simulink model "MVC27_Sim"  (R2022b)
settings: Solver=FixedStepAuto  StartTime=0.0  StopTime=Sim.Tsim  FixedStep=Sim.Ts  RelTol=1e-3
values from neighbouring files (symbols this model uses):
  g = 9.81    [sim_para.m]
  tdis_FL = 0.3455    [meso_para.m]
  tdis_FR = 0.3455    [meso_para.m]
  tdis_RL = 1 - (tdis_FR + tdis_FL + tdis_RR)    (= 0.1545)    [meso_para.m]
  tdis_RR = 0.1545    [meso_para.m]
undefined symbols (not defined in the file or in its folder): Ctl, DYC, EPS, flag, Motor, Road, Sim, Slip, Steer, Vehicle, Wheel, Wind, WPT
libraries: simulink x3
(part 2 of 2)

== system MVC27_Sim/Energy Management & Motion Control Strategy/Steer angle and yaw moment control/steering angle control ==
  POS_Y : Inport
  Yaw : Inport  Port=2
  Add : Sum  Inputs=+-
  Add1 : Sum  Inputs=+-
  Add2 : Sum
  Constant : Constant  Value=0
  Constant1 : Constant  Value=0
  Position control gain : Gain  Gain=Steer.Kp_pos
  Yaw control gain : Gain  Gain=Steer.Kp_yaw
  delta_f_cmd : Outport
  wires:
  Constant/1 -> Add/1
  POS_Y/1 -> Add/2
  Add/1 -> Position control gain/1
  Constant1/1 -> Add1/1
  Yaw/1 -> Add1/2
  Add1/1 -> Yaw control gain/1
  Position control gain/1 -> Add2/1
  Yaw control gain/1 -> Add2/2
  Add2/1 -> delta_f_cmd/1

== system MVC27_Sim/Energy Management & Motion Control Strategy/Steer angle and yaw moment control/yaw moment control_pos_y ==
  In1 : Inport
  Add : Sum  Inputs=+-
  Add1 : Sum  Inputs=+++
  Constant : Constant  Value=0
  Gain1 : Gain  Gain=DYC.Kd_pos
  Gain2 : Gain  Gain=DYC.Kp_pos
  Gain3 : Gain  Gain=DYC.Ki_pos
  Integrator : Integrator
  Transfer Fcn : TransferFcn  Numerator=[1 0]  Denominator=[DYC.Taud_pos 1]
  Out1 : Outport
  wires:
  Gain2/1 -> Add1/1
  Add1/1 -> Out1/1
  Integrator/1 -> Add1/2
  Transfer Fcn/1 -> Add1/3
  Gain1/1 -> Transfer Fcn/1
  Gain3/1 -> Integrator/1
  Constant/1 -> Add/1
  Add/1 -> Gain1/1, Gain2/1, Gain3/1
  In1/1 -> Add/2

== system MVC27_Sim/Energy Management & Motion Control Strategy/Steer angle and yaw moment control/yaw moment control_yaw ==
  In1 : Inport
  Add : Sum  Inputs=+-
  Constant : Constant  Value=0
  Gain3 : Gain  Gain=DYC.Kp_yaw
  Out1 : Outport
  wires:
  Gain3/1 -> Out1/1
  Constant/1 -> Add/1
  Add/1 -> Gain3/1
  In1/1 -> Add/2

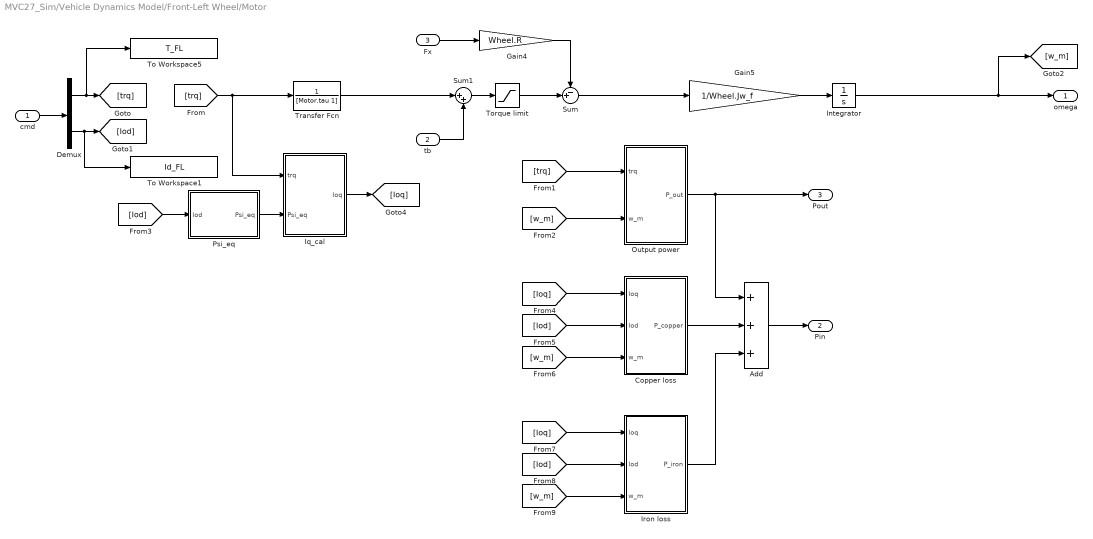
== system MVC27_Sim/Vehicle Dynamics Model/Front-Left Wheel/Motor ==
  cmd : Inport
  tb : Inport  Port=2
  Fx : Inport  Port=3
  Add : Sum  Inputs=+++
  Copper loss : Subsystem
  Demux : Demux  Outputs=2
  Gain4 : Gain  Gain=Wheel.R  SaturateOnIntegerOverflow=on  OutDataTypeStr=Inherit: Same as input  ParamDataTypeStr=Inherit: Same as input
  Gain5 : Gain  Gain=1/Wheel.Jw_f  SaturateOnIntegerOverflow=on  OutDataTypeStr=Inherit: Same as input  ParamDataTypeStr=Inherit: Same as input
  Integrator : Integrator  InitialCondition=Sim.Ini_W  LowerSaturationLimit=0
  Iq_cal : Subsystem
  Iron loss : Subsystem
  Output power : Subsystem
  Psi_eq : Subsystem
  Sum : Sum  Inputs=-+|  SaturateOnIntegerOverflow=on
  Sum1 : Sum  Inputs=|++
  To Workspace1 : ToWorkspace  VariableName=Id_FL  SampleTime=-1
  To Workspace5 : ToWorkspace  VariableName=T_FL  SampleTime=-1
  Torque limit : Saturate  UpperLimit=Motor.Tmax_f  LowerLimit=-Motor.Tmax_f
  Transfer Fcn : TransferFcn  Denominator=[Motor.tau 1]
  omega : Outport
  Pin : Outport  Port=2
  Pout : Outport  Port=3
  wires:
  Gain4/1 -> Sum/1
  Gain5/1 -> Integrator/1
  Sum/1 -> Gain5/1
  Torque limit/1 -> Sum/2
  cmd/1 -> Demux/1
  Demux/1 -> To Workspace5/1, [trq]
  Sum1/1 -> Torque limit/1
  tb/1 -> Sum1/2
  Demux/2 -> To Workspace1/1, [Iod]
  Fx/1 -> Gain4/1
  [trq] -> Output power/1(trq)
  [w_m] -> Output power/2(w_m)
  Iq_cal/1(Ioq) -> [Ioq]
  [Iod] -> Psi_eq/1(Iod)
  Psi_eq/1(Psi_eq) -> Iq_cal/2(Psi_eq)
  [Ioq] -> Copper loss/1(Ioq)
  [Iod] -> Copper loss/2(Iod)
  [w_m] -> Copper loss/3(w_m)
  [Ioq] -> Iron loss/1(Ioq)
  [Iod] -> Iron loss/2(Iod)
  [w_m] -> Iron loss/3(w_m)
  Copper loss/1(P_copper) -> Add/2
  Output power/1(P_out) -> Pout/1, Add/1
  Iron loss/1(P_iron) -> Add/3
  Add/1 -> Pin/1
  Integrator/1 -> omega/1, [w_m]
  [trq] -> Transfer Fcn/1, Iq_cal/1(trq)
  Transfer Fcn/1 -> Sum1/1

== system MVC27_Sim/Vehicle Dynamics Model/Front-Left Wheel/Tire force model ==
  V : Inport
  Vw : Inport  Port=2
  alpha : Inport  Port=3
  mu : Inport  Port=4
  Fz : Inport  Port=5
  Demux : Demux  Outputs=3
      settings: DisplayOption=none
  Level-2 MATLAB S-Function : M-S-Function  FunctionName=LambdaMethod
  Mux : Mux  Inputs=5
  Slip ratio calculation : Subsystem
  Transfer Fcn : TransferFcn  Denominator=[0.01 1]
  Transfer Fcn1 : TransferFcn  Denominator=[0.01 1]
  Transfer Fcn2 : TransferFcn  Denominator=[0.01 1]
  lambda_cal : Scope
  Fx : Outport
  Fy : Outport  Port=2
  lambda : Outport  Port=3
  wires:
  V/1 -> Slip ratio calculation/1(V), Mux/1
  Demux/2 -> Transfer Fcn1/1
  Demux/3 -> Transfer Fcn2/1
  Vw/1 -> Slip ratio calculation/2(Vw), Mux/2
  Mux/1 -> Level-2 MATLAB S-Function/1
  mu/1 -> Mux/4
  Demux/1 -> Transfer Fcn/1
  Fz/1 -> Mux/5
  alpha/1 -> Mux/3
  Slip ratio calculation/1(lambda) -> lambda_cal/1
  Transfer Fcn/1 -> Fx/1
  Transfer Fcn1/1 -> Fy/1
  Transfer Fcn2/1 -> lambda/1
  Level-2 MATLAB S-Function/1 -> Demux/1

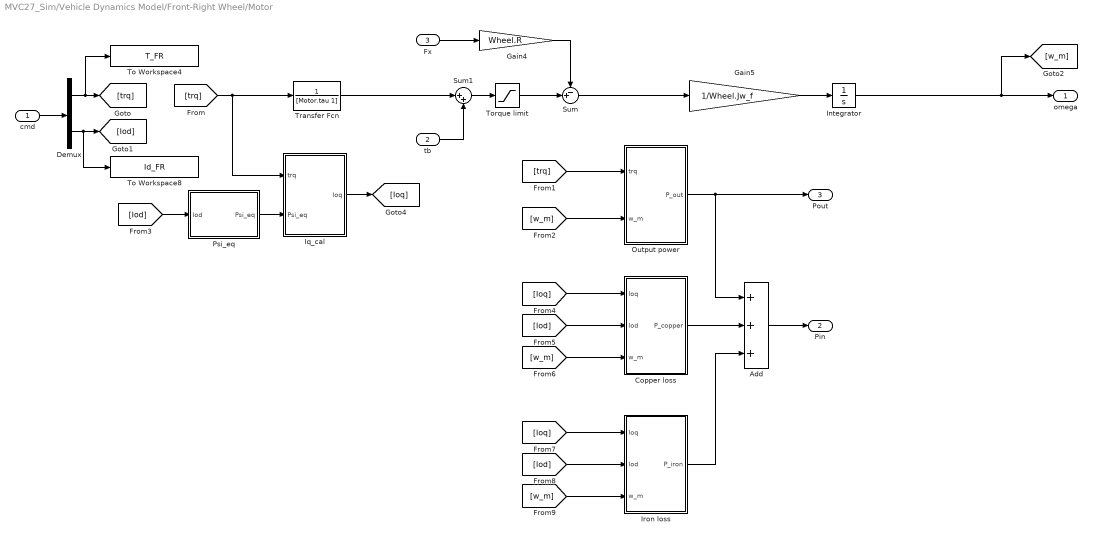
== system MVC27_Sim/Vehicle Dynamics Model/Front-Right Wheel/Motor ==
  cmd : Inport
  tb : Inport  Port=2
  Fx : Inport  Port=3
  Add : Sum  Inputs=+++
  Copper loss : Subsystem
  Demux : Demux  Outputs=2
  Gain4 : Gain  Gain=Wheel.R  SaturateOnIntegerOverflow=on  OutDataTypeStr=Inherit: Same as input  ParamDataTypeStr=Inherit: Same as input
  Gain5 : Gain  Gain=1/Wheel.Jw_f  SaturateOnIntegerOverflow=on  OutDataTypeStr=Inherit: Same as input  ParamDataTypeStr=Inherit: Same as input
  Integrator : Integrator  InitialCondition=Sim.Ini_W  LowerSaturationLimit=0
  Iq_cal : Subsystem
  Iron loss : Subsystem
  Output power : Subsystem
  Psi_eq : Subsystem
  Sum : Sum  Inputs=-+|  SaturateOnIntegerOverflow=on
  Sum1 : Sum  Inputs=|++
  To Workspace4 : ToWorkspace  VariableName=T_FR  SampleTime=-1
  To Workspace8 : ToWorkspace  VariableName=Id_FR  SampleTime=-1
  Torque limit : Saturate  UpperLimit=Motor.Tmax_f  LowerLimit=-Motor.Tmax_f
  Transfer Fcn : TransferFcn  Denominator=[Motor.tau 1]
  omega : Outport
  Pin : Outport  Port=2
  Pout : Outport  Port=3
  wires:
  Gain4/1 -> Sum/1
  Gain5/1 -> Integrator/1
  Sum/1 -> Gain5/1
  Torque limit/1 -> Sum/2
  cmd/1 -> Demux/1
  Demux/1 -> To Workspace4/1, [trq]
  Sum1/1 -> Torque limit/1
  tb/1 -> Sum1/2
  Demux/2 -> To Workspace8/1, [Iod]
  Fx/1 -> Gain4/1
  [trq] -> Output power/1(trq)
  [w_m] -> Output power/2(w_m)
  Iq_cal/1(Ioq) -> [Ioq]
  [Iod] -> Psi_eq/1(Iod)
  Psi_eq/1(Psi_eq) -> Iq_cal/2(Psi_eq)
  [Ioq] -> Copper loss/1(Ioq)
  [Iod] -> Copper loss/2(Iod)
  [w_m] -> Copper loss/3(w_m)
  [Ioq] -> Iron loss/1(Ioq)
  [Iod] -> Iron loss/2(Iod)
  [w_m] -> Iron loss/3(w_m)
  Copper loss/1(P_copper) -> Add/2
  Output power/1(P_out) -> Pout/1, Add/1
  Iron loss/1(P_iron) -> Add/3
  Add/1 -> Pin/1
  Integrator/1 -> omega/1, [w_m]
  [trq] -> Transfer Fcn/1, Iq_cal/1(trq)
  Transfer Fcn/1 -> Sum1/1

== system MVC27_Sim/Vehicle Dynamics Model/Front-Right Wheel/Tire force model ==
  V : Inport
  Vw : Inport  Port=2
  alpha : Inport  Port=3
  mu : Inport  Port=4
  Fz : Inport  Port=5
  Demux : Demux  Outputs=3
      settings: DisplayOption=none
  Level-2 MATLAB S-Function : M-S-Function  FunctionName=LambdaMethod
  Mux : Mux  Inputs=5
  Slip ratio calculation : Subsystem
  Transfer Fcn : TransferFcn  Denominator=[0.01 1]
  Transfer Fcn1 : TransferFcn  Denominator=[0.01 1]
  Transfer Fcn2 : TransferFcn  Denominator=[0.01 1]
  lambda_cal : Scope
  Fx : Outport
  Fy : Outport  Port=2
  lambda : Outport  Port=3
  wires:
  V/1 -> Slip ratio calculation/1(V), Mux/1
  Demux/2 -> Transfer Fcn1/1
  Demux/3 -> Transfer Fcn2/1
  Vw/1 -> Slip ratio calculation/2(Vw), Mux/2
  Mux/1 -> Level-2 MATLAB S-Function/1
  mu/1 -> Mux/4
  Demux/1 -> Transfer Fcn/1
  Fz/1 -> Mux/5
  alpha/1 -> Mux/3
  Slip ratio calculation/1(lambda) -> lambda_cal/1
  Transfer Fcn/1 -> Fx/1
  Transfer Fcn1/1 -> Fy/1
  Transfer Fcn2/1 -> lambda/1
  Level-2 MATLAB S-Function/1 -> Demux/1

== system MVC27_Sim/Vehicle Dynamics Model/Rear-Left Wheel/Motor ==
  cmd : Inport
  tb : Inport  Port=2
  Fx : Inport  Port=3
  Add : Sum  Inputs=+++
  Copper loss : Subsystem
  Demux : Demux  Outputs=2
  Gain4 : Gain  Gain=Wheel.R  SaturateOnIntegerOverflow=on  OutDataTypeStr=Inherit: Same as input  ParamDataTypeStr=Inherit: Same as input
  Gain5 : Gain  Gain=1/Wheel.Jw_r  SaturateOnIntegerOverflow=on  OutDataTypeStr=Inherit: Same as input  ParamDataTypeStr=Inherit: Same as input
  Integrator : Integrator  InitialCondition=Sim.Ini_W  LowerSaturationLimit=0
  Iq_cal : Subsystem
  Iron loss : Subsystem
  Output power : Subsystem
  Psi_eq : Subsystem
  Sum : Sum  Inputs=-+|  SaturateOnIntegerOverflow=on
  Sum1 : Sum  Inputs=|++
  To Workspace3 : ToWorkspace  VariableName=Id_RL  SampleTime=-1
  To Workspace7 : ToWorkspace  VariableName=T_RL  SampleTime=-1
  Torque limit : Saturate  UpperLimit=Motor.Tmax_r  LowerLimit=-Motor.Tmax_r
  Transfer Fcn : TransferFcn  Denominator=[Motor.tau 1]
  omega : Outport
  Pin : Outport  Port=2
  Pout : Outport  Port=3
  wires:
  Gain4/1 -> Sum/1
  Gain5/1 -> Integrator/1
  Sum/1 -> Gain5/1
  Torque limit/1 -> Sum/2
  cmd/1 -> Demux/1
  Demux/1 -> To Workspace7/1, [trq]
  [trq] -> Transfer Fcn/1, Iq_cal/1(trq)
  Sum1/1 -> Torque limit/1
  tb/1 -> Sum1/2
  Demux/2 -> To Workspace3/1, [Iod]
  Fx/1 -> Gain4/1
  [trq] -> Output power/1(trq)
  [w_m] -> Output power/2(w_m)
  Iq_cal/1(Ioq) -> [Ioq]
  [Iod] -> Psi_eq/1(Iod)
  Psi_eq/1(Psi_eq) -> Iq_cal/2(Psi_eq)
  [Ioq] -> Copper loss/1(Ioq)
  [Iod] -> Copper loss/2(Iod)
  [w_m] -> Copper loss/3(w_m)
  [Ioq] -> Iron loss/1(Ioq)
  [Iod] -> Iron loss/2(Iod)
  [w_m] -> Iron loss/3(w_m)
  Copper loss/1(P_copper) -> Add/2
  Output power/1(P_out) -> Pout/1, Add/1
  Iron loss/1(P_iron) -> Add/3
  Add/1 -> Pin/1
  Integrator/1 -> omega/1, [w_m]
  Transfer Fcn/1 -> Sum1/1

== system MVC27_Sim/Vehicle Dynamics Model/Rear-Left Wheel/Tire force model ==
  V : Inport
  Vw : Inport  Port=2
  alpha : Inport  Port=3
  mu : Inport  Port=4
  Fz : Inport  Port=5
  Demux : Demux  Outputs=3
      settings: DisplayOption=none
  Level-2 MATLAB S-Function : M-S-Function  FunctionName=LambdaMethod
  Mux : Mux  Inputs=5
  Slip ratio calculation : Subsystem
  Transfer Fcn : TransferFcn  Denominator=[0.01 1]
  Transfer Fcn1 : TransferFcn  Denominator=[0.01 1]
  Transfer Fcn2 : TransferFcn  Denominator=[0.01 1]
  lambda_cal : Scope
  Fx : Outport
  Fy : Outport  Port=2
  lambda : Outport  Port=3
  wires:
  V/1 -> Slip ratio calculation/1(V), Mux/1
  Demux/3 -> Transfer Fcn2/1
  Vw/1 -> Slip ratio calculation/2(Vw), Mux/2
  mu/1 -> Mux/4
  Demux/1 -> Transfer Fcn/1
  Fz/1 -> Mux/5
  alpha/1 -> Mux/3
  Slip ratio calculation/1(lambda) -> lambda_cal/1
  Demux/2 -> Transfer Fcn1/1
  Transfer Fcn/1 -> Fx/1
  Transfer Fcn1/1 -> Fy/1
  Transfer Fcn2/1 -> lambda/1
  Mux/1 -> Level-2 MATLAB S-Function/1
  Level-2 MATLAB S-Function/1 -> Demux/1

== system MVC27_Sim/Vehicle Dynamics Model/Rear-Right Wheel/Motor ==
  cmd : Inport
  tb : Inport  Port=2
  Fx : Inport  Port=3
  Add : Sum  Inputs=+++
  Copper loss : Subsystem
  Demux : Demux  Outputs=2
  Gain4 : Gain  Gain=Wheel.R  SaturateOnIntegerOverflow=on  OutDataTypeStr=Inherit: Same as input  ParamDataTypeStr=Inherit: Same as input
  Gain5 : Gain  Gain=1/Wheel.Jw_r  SaturateOnIntegerOverflow=on  OutDataTypeStr=Inherit: Same as input  ParamDataTypeStr=Inherit: Same as input
  Integrator : Integrator  InitialCondition=Sim.Ini_W  LowerSaturationLimit=0
  Iq_cal : Subsystem
  Iron loss : Subsystem
  Output power : Subsystem
  Psi_eq : Subsystem
  Sum : Sum  Inputs=-+|  SaturateOnIntegerOverflow=on
  Sum1 : Sum  Inputs=|++
  To Workspace2 : ToWorkspace  VariableName=Id_RR  SampleTime=-1
  To Workspace6 : ToWorkspace  VariableName=T_RR  SampleTime=-1
  Torque limit : Saturate  UpperLimit=Motor.Tmax_r  LowerLimit=-Motor.Tmax_r
  Transfer Fcn : TransferFcn  Denominator=[Motor.tau 1]
  omega : Outport
  Pin : Outport  Port=2
  Pout : Outport  Port=3
  wires:
  Gain4/1 -> Sum/1
  Gain5/1 -> Integrator/1
  Sum/1 -> Gain5/1
  Torque limit/1 -> Sum/2
  cmd/1 -> Demux/1
  Demux/1 -> To Workspace6/1, [trq]
  Sum1/1 -> Torque limit/1
  tb/1 -> Sum1/2
  Demux/2 -> To Workspace2/1, [Iod]
  Fx/1 -> Gain4/1
  [trq] -> Output power/1(trq)
  [w_m] -> Output power/2(w_m)
  Iq_cal/1(Ioq) -> [Ioq]
  [Iod] -> Psi_eq/1(Iod)
  Psi_eq/1(Psi_eq) -> Iq_cal/2(Psi_eq)
  [Ioq] -> Copper loss/1(Ioq)
  [Iod] -> Copper loss/2(Iod)
  [w_m] -> Copper loss/3(w_m)
  [Ioq] -> Iron loss/1(Ioq)
  [Iod] -> Iron loss/2(Iod)
  [w_m] -> Iron loss/3(w_m)
  Copper loss/1(P_copper) -> Add/2
  Output power/1(P_out) -> Pout/1, Add/1
  Iron loss/1(P_iron) -> Add/3
  Add/1 -> Pin/1
  Integrator/1 -> omega/1, [w_m]
  [trq] -> Transfer Fcn/1, Iq_cal/1(trq)
  Transfer Fcn/1 -> Sum1/1

== system MVC27_Sim/Vehicle Dynamics Model/Rear-Right Wheel/Tire force model ==
  V : Inport
  Vw : Inport  Port=2
  alpha : Inport  Port=3
  mu : Inport  Port=4
  Fz : Inport  Port=5
  Demux : Demux  Outputs=3
      settings: DisplayOption=none
  Level-2 MATLAB S-Function : M-S-Function  FunctionName=LambdaMethod
  Mux : Mux  Inputs=5
  Slip ratio calculation : Subsystem
  Transfer Fcn : TransferFcn  Denominator=[0.01 1]
  Transfer Fcn1 : TransferFcn  Denominator=[0.01 1]
  Transfer Fcn2 : TransferFcn  Denominator=[0.01 1]
  lambda_cal : Scope
  Fx : Outport
  Fy : Outport  Port=2
  lambda : Outport  Port=3
  wires:
  V/1 -> Slip ratio calculation/1(V), Mux/1
  Demux/2 -> Transfer Fcn1/1
  Demux/3 -> Transfer Fcn2/1
  Vw/1 -> Slip ratio calculation/2(Vw), Mux/2
  Mux/1 -> Level-2 MATLAB S-Function/1
  mu/1 -> Mux/4
  Demux/1 -> Transfer Fcn/1
  Fz/1 -> Mux/5
  alpha/1 -> Mux/3
  Slip ratio calculation/1(lambda) -> lambda_cal/1
  Transfer Fcn/1 -> Fx/1
  Transfer Fcn1/1 -> Fy/1
  Transfer Fcn2/1 -> lambda/1
  Level-2 MATLAB S-Function/1 -> Demux/1

== system MVC27_Sim/Vehicle Dynamics Model/Vehicle Body/Condition to prevent division by zero ==
  In : Inport
  Constant : Constant  Value=0.1
  Scope : Scope
  Switch : Switch  Criteria=u2 > Threshold  Threshold=0.1  SaturateOnIntegerOverflow=off  InputSameDT=off
  Out : Outport
  wires:
  In/1 -> Switch/1, Switch/2
  Constant/1 -> Switch/3
  Switch/1 -> Scope/1, Out/1

== system MVC27_Sim/Vehicle Dynamics Model/Vehicle Body/Driving resistance ==
  Vx : Inport
  Abs : Abs  SaturateOnIntegerOverflow=off
  Air resistance : Constant  Value=1/2*Vehicle.rho*Vehicle.Cd*Vehicle.Afpa
  Memory1 : Memory  InheritSampleTime=on  LinearizeMemory=on
  Plus1 : Sum
  Product : Product  Inputs=3
  Rolling resistance : Constant  Value=Vehicle.mu0*Vehicle.M*g
  DR : Outport
  wires:
  Product/1 -> Plus1/2
  Air resistance/1 -> Product/1
  Plus1/1 -> DR/1
  Vx/1 -> Memory1/1
  Memory1/1 -> Product/2, Abs/1
  Abs/1 -> Product/3
  Rolling resistance/1 -> Plus1/1

== system MVC27_Sim/Vehicle Dynamics Model/Vehicle Body/Lateral disturbance ==
  Wind_flag : Inport
  Clock{,1..3} (4 alike) : Clock
  Product : Product
  Product1 : Product
  Switch : Switch  Criteria=u2 > Threshold  Threshold=Wind.time_start  SaturateOnIntegerOverflow=off  InputSameDT=off
  Switch1 : Switch  Criteria=u2 > Threshold  Threshold=Wind.time_stop  SaturateOnIntegerOverflow=off  InputSameDT=off
  Switch2 : Switch  Criteria=u2 > Threshold  Threshold=Wind.time_start  SaturateOnIntegerOverflow=off  InputSameDT=off
  Switch3 : Switch  Criteria=u2 > Threshold  Threshold=Wind.time_stop  SaturateOnIntegerOverflow=off  InputSameDT=off
  Wind force : Scope
  Wind force.No : Constant  Value=0
  Wind force.Yes : Constant  Value=Wind.force
  Wind moment : Scope
  Wind moment.No : Constant  Value=0
  Wind moment.Yes : Constant  Value=Wind.moment
  Nzd : Outport
  Fyd : Outport  Port=2
  wires:
  Clock/1 -> Switch/2
  Clock1/1 -> Switch1/2
  Wind force.Yes/1 -> Switch/1
  Wind force.No/1 -> Switch1/1, Switch/3
  Switch/1 -> Switch1/3
  Switch2/1 -> Switch3/3
  Clock2/1 -> Switch2/2
  Wind moment.Yes/1 -> Switch2/1
  Clock3/1 -> Switch3/2
  Wind moment.No/1 -> Switch3/1, Switch2/3
  Switch3/1 -> Product/1
  Switch1/1 -> Product1/2
  Product1/1 -> Wind force/1, Fyd/1
  Product/1 -> Wind moment/1, Nzd/1
  Wind_flag/1 -> Product1/1, Product/2

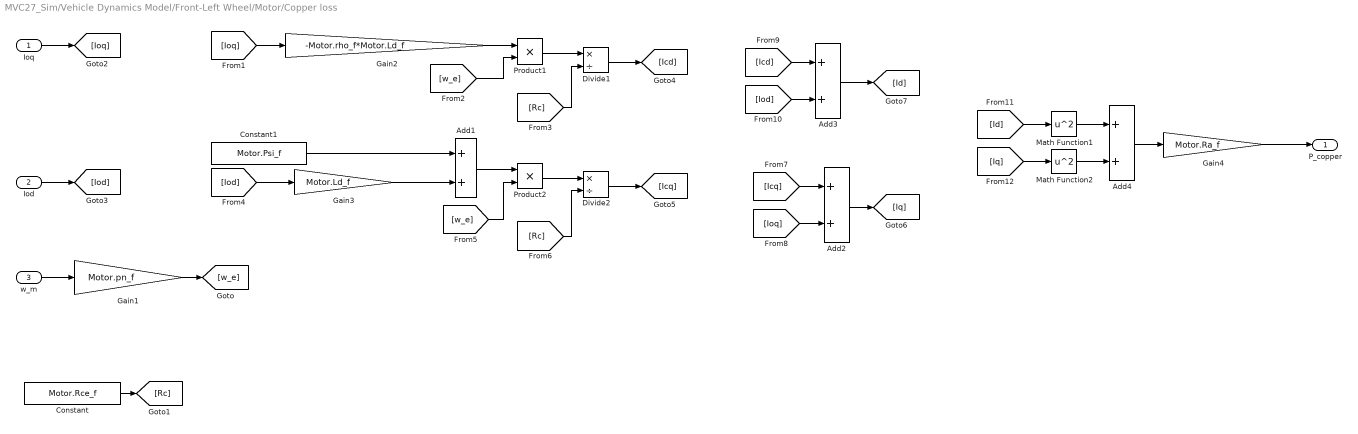
== system MVC27_Sim/Vehicle Dynamics Model/Front-Left Wheel/Motor/Copper loss ==
  Ioq : Inport
  Iod : Inport  Port=2
  w_m : Inport  Port=3
  Add{1..4} (4 alike) : Sum
  Constant : Constant  Value=Motor.Rce_f
  Constant1 : Constant  Value=Motor.Psi_f
  Divide1 : Product  Inputs=*/
  Divide2 : Product  Inputs=*/
  Gain1 : Gain  Gain=Motor.pn_f
  Gain2 : Gain  Gain=-Motor.rho_f*Motor.Ld_f
  Gain3 : Gain  Gain=Motor.Ld_f
  Gain4 : Gain  Gain=Motor.Ra_f
  Math Function1 : Math  Operator=square  SignedPower=on
  Math Function2 : Math  Operator=square  SignedPower=on
  Product1 : Product
  Product2 : Product
  P_copper : Outport
  wires:
  w_m/1 -> Gain1/1
  Gain1/1 -> [w_e]
  Ioq/1 -> [Ioq]
  Iod/1 -> [Iod]
  [Ioq] -> Gain2/1
  Gain2/1 -> Product1/1
  [w_e] -> Product1/2
  Product1/1 -> Divide1/1
  [Rc] -> Divide1/2
  Divide1/1 -> [Icd]
  Constant1/1 -> Add1/1
  [Iod] -> Gain3/1
  Gain3/1 -> Add1/2
  Add1/1 -> Product2/1
  [w_e] -> Product2/2
  Product2/1 -> Divide2/1
  [Rc] -> Divide2/2
  Divide2/1 -> [Icq]
  [Icq] -> Add2/1
  [Ioq] -> Add2/2
  Add2/1 -> [Iq]
  [Icd] -> Add3/1
  Add3/1 -> [Id]
  [Iod] -> Add3/2
  [Id] -> Math Function1/1
  [Iq] -> Math Function2/1
  Math Function1/1 -> Add4/1
  Math Function2/1 -> Add4/2
  Add4/1 -> Gain4/1
  Gain4/1 -> P_copper/1
  Constant/1 -> [Rc]

== system MVC27_Sim/Vehicle Dynamics Model/Front-Left Wheel/Motor/Iq_cal ==
  trq : Inport
  Psi_eq : Inport  Port=2
  Divide : Product  Inputs=*/
  Gain : Gain  Gain=Motor.pn_f
  Ioq : Outport
  wires:
  Gain/1 -> Divide/2
  Divide/1 -> Ioq/1
  Psi_eq/1 -> Gain/1
  trq/1 -> Divide/1

== system MVC27_Sim/Vehicle Dynamics Model/Front-Left Wheel/Motor/Iron loss ==
  Ioq : Inport
  Iod : Inport  Port=2
  w_m : Inport  Port=3
  Add1 : Sum
  Add4 : Sum
  Constant : Constant  Value=Motor.Rce_f
  Constant1 : Constant  Value=Motor.Psi_f
  Divide1 : Product  Inputs=*/
  Divide2 : Product  Inputs=*/
  Gain1 : Gain  Gain=Motor.pn_f
  Gain2 : Gain  Gain=-Motor.rho_f*Motor.Ld_f
  Gain3 : Gain  Gain=Motor.Ld_f
  Math Function1 : Math  Operator=square  SignedPower=on
  Math Function2 : Math  Operator=square  SignedPower=on
  Product1 : Product
  Product2 : Product
  Product3 : Product
  P_iron : Outport
  wires:
  Gain1/1 -> [w_e]
  w_m/1 -> Gain1/1
  [Rc] -> Divide2/2
  Constant1/1 -> Add1/1
  Gain3/1 -> Add1/2
  Add1/1 -> Product2/1
  Divide1/1 -> [Icd]
  Product1/1 -> Divide1/1
  [Iod] -> Gain3/1
  Gain2/1 -> Product1/1
  Divide2/1 -> [Icq]
  [Rc] -> Divide1/2
  [Ioq] -> Gain2/1
  [w_e] -> Product2/2
  [w_e] -> Product1/2
  Product2/1 -> Divide2/1
  Ioq/1 -> [Ioq]
  Iod/1 -> [Iod]
  [Icd] -> Math Function1/1
  Math Function1/1 -> Add4/1
  [Icq] -> Math Function2/1
  Math Function2/1 -> Add4/2
  Add4/1 -> Product3/1
  [Rc] -> Product3/2
  Product3/1 -> P_iron/1
  Constant/1 -> [Rc]

== system MVC27_Sim/Vehicle Dynamics Model/Front-Left Wheel/Motor/Output power ==
  trq : Inport
  w_m : Inport  Port=2
  Product : Product
  P_out : Outport
  wires:
  trq/1 -> Product/1
  w_m/1 -> Product/2
  Product/1 -> P_out/1

== system MVC27_Sim/Vehicle Dynamics Model/Front-Left Wheel/Motor/Psi_eq ==
  Iod : Inport
  Add : Sum
  Constant : Constant  Value=Motor.Psi_f
  Gain4 : Gain  Gain=(1-Motor.rho_f)*Motor.Ld_f  SaturateOnIntegerOverflow=on  OutDataTypeStr=Inherit: Same as input  ParamDataTypeStr=Inherit: Same as input
  Psi_eq : Outport
  wires:
  Iod/1 -> Gain4/1
  Gain4/1 -> Add/2
  Constant/1 -> Add/1
  Add/1 -> Psi_eq/1

== system MVC27_Sim/Vehicle Dynamics Model/Front-Left Wheel/Tire force model/Slip ratio calculation ==
  V : Inport
  Vw : Inport  Port=2
  Divide : Product  Inputs=*/
  Sum : Sum  Inputs=-+
  max calculation : MinMax  Function=max  Inputs=2
  max calculation1 : MinMax  Function=max  Inputs=2
  small number for anti division by zero : Constant  Value=eps
  lambda : Outport
  wires:
  small number for anti division by zero/1 -> max calculation1/2
  Vw/1 -> max calculation/2, Sum/2
  V/1 -> max calculation/1, Sum/1
  Divide/1 -> lambda/1
  max calculation/1 -> max calculation1/1
  max calculation1/1 -> Divide/2
  Sum/1 -> Divide/1

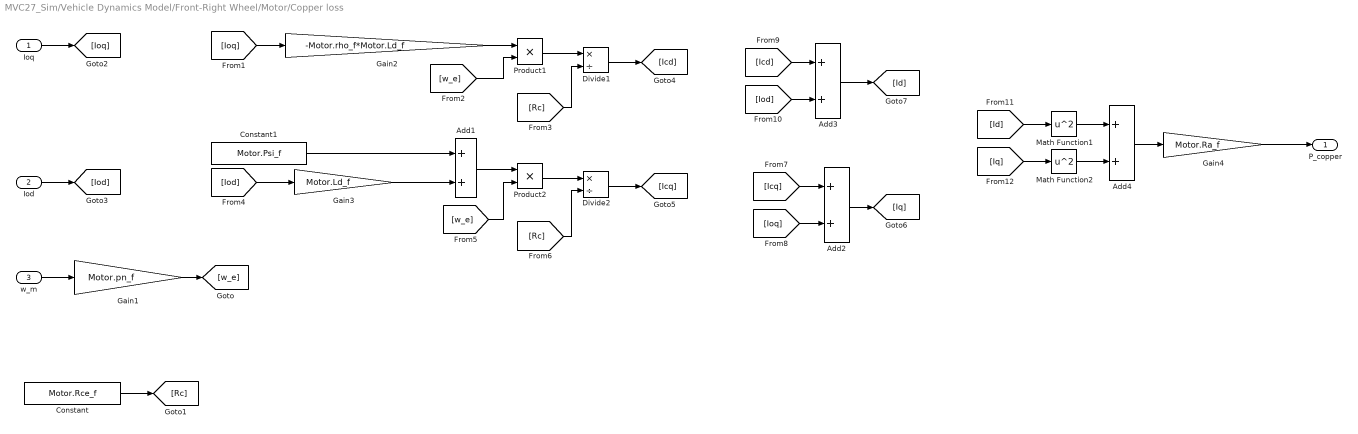
== system MVC27_Sim/Vehicle Dynamics Model/Front-Right Wheel/Motor/Copper loss ==
  Ioq : Inport
  Iod : Inport  Port=2
  w_m : Inport  Port=3
  Add{1..4} (4 alike) : Sum
  Constant : Constant  Value=Motor.Rce_f
  Constant1 : Constant  Value=Motor.Psi_f
  Divide1 : Product  Inputs=*/
  Divide2 : Product  Inputs=*/
  Gain1 : Gain  Gain=Motor.pn_f
  Gain2 : Gain  Gain=-Motor.rho_f*Motor.Ld_f
  Gain3 : Gain  Gain=Motor.Ld_f
  Gain4 : Gain  Gain=Motor.Ra_f
  Math Function1 : Math  Operator=square  SignedPower=on
  Math Function2 : Math  Operator=square  SignedPower=on
  Product1 : Product
  Product2 : Product
  P_copper : Outport
  wires:
  w_m/1 -> Gain1/1
  Gain1/1 -> [w_e]
  Ioq/1 -> [Ioq]
  Iod/1 -> [Iod]
  [Ioq] -> Gain2/1
  Gain2/1 -> Product1/1
  [w_e] -> Product1/2
  Product1/1 -> Divide1/1
  [Rc] -> Divide1/2
  Divide1/1 -> [Icd]
  Constant1/1 -> Add1/1
  [Iod] -> Gain3/1
  Gain3/1 -> Add1/2
  Add1/1 -> Product2/1
  [w_e] -> Product2/2
  Product2/1 -> Divide2/1
  [Rc] -> Divide2/2
  Divide2/1 -> [Icq]
  [Icq] -> Add2/1
  [Ioq] -> Add2/2
  Add2/1 -> [Iq]
  [Icd] -> Add3/1
  Add3/1 -> [Id]
  [Iod] -> Add3/2
  [Id] -> Math Function1/1
  [Iq] -> Math Function2/1
  Math Function1/1 -> Add4/1
  Math Function2/1 -> Add4/2
  Add4/1 -> Gain4/1
  Gain4/1 -> P_copper/1
  Constant/1 -> [Rc]

== system MVC27_Sim/Vehicle Dynamics Model/Front-Right Wheel/Motor/Iq_cal ==
  trq : Inport
  Psi_eq : Inport  Port=2
  Divide : Product  Inputs=*/
  Gain : Gain  Gain=Motor.pn_f
  Ioq : Outport
  wires:
  Psi_eq/1 -> Gain/1
  Gain/1 -> Divide/2
  trq/1 -> Divide/1
  Divide/1 -> Ioq/1

== system MVC27_Sim/Vehicle Dynamics Model/Front-Right Wheel/Motor/Iron loss ==
  Ioq : Inport
  Iod : Inport  Port=2
  w_m : Inport  Port=3
  Add1 : Sum
  Add4 : Sum
  Constant : Constant  Value=Motor.Rce_f
  Constant1 : Constant  Value=Motor.Psi_f
  Divide1 : Product  Inputs=*/
  Divide2 : Product  Inputs=*/
  Gain1 : Gain  Gain=Motor.pn_f
  Gain2 : Gain  Gain=-Motor.rho_f*Motor.Ld_f
  Gain3 : Gain  Gain=Motor.Ld_f
  Math Function1 : Math  Operator=square  SignedPower=on
  Math Function2 : Math  Operator=square  SignedPower=on
  Product1 : Product
  Product2 : Product
  Product3 : Product
  P_iron : Outport
  wires:
  Gain1/1 -> [w_e]
  w_m/1 -> Gain1/1
  [Rc] -> Divide2/2
  Constant1/1 -> Add1/1
  Gain3/1 -> Add1/2
  Add1/1 -> Product2/1
  Divide1/1 -> [Icd]
  Product1/1 -> Divide1/1
  [Iod] -> Gain3/1
  Gain2/1 -> Product1/1
  Divide2/1 -> [Icq]
  [Rc] -> Divide1/2
  [Ioq] -> Gain2/1
  [w_e] -> Product2/2
  [w_e] -> Product1/2
  Product2/1 -> Divide2/1
  Ioq/1 -> [Ioq]
  Iod/1 -> [Iod]
  [Icd] -> Math Function1/1
  Math Function1/1 -> Add4/1
  [Icq] -> Math Function2/1
  Math Function2/1 -> Add4/2
  Add4/1 -> Product3/1
  [Rc] -> Product3/2
  Product3/1 -> P_iron/1
  Constant/1 -> [Rc]

== system MVC27_Sim/Vehicle Dynamics Model/Front-Right Wheel/Motor/Output power ==
  trq : Inport
  w_m : Inport  Port=2
  Product : Product
  P_out : Outport
  wires:
  trq/1 -> Product/1
  w_m/1 -> Product/2
  Product/1 -> P_out/1

== system MVC27_Sim/Vehicle Dynamics Model/Front-Right Wheel/Motor/Psi_eq ==
  Iod : Inport
  Add : Sum
  Constant : Constant  Value=Motor.Psi_f
  Gain4 : Gain  Gain=(1-Motor.rho_f)*Motor.Ld_f  SaturateOnIntegerOverflow=on  OutDataTypeStr=Inherit: Same as input  ParamDataTypeStr=Inherit: Same as input
  Psi_eq : Outport
  wires:
  Iod/1 -> Gain4/1
  Gain4/1 -> Add/2
  Constant/1 -> Add/1
  Add/1 -> Psi_eq/1

== system MVC27_Sim/Vehicle Dynamics Model/Front-Right Wheel/Tire force model/Slip ratio calculation ==
  V : Inport
  Vw : Inport  Port=2
  Divide : Product  Inputs=*/
  Sum : Sum  Inputs=-+
  max calculation : MinMax  Function=max  Inputs=2
  max calculation1 : MinMax  Function=max  Inputs=2
  small number for anti division by zero : Constant  Value=eps
  lambda : Outport
  wires:
  small number for anti division by zero/1 -> max calculation1/2
  Vw/1 -> max calculation/2, Sum/2
  V/1 -> max calculation/1, Sum/1
  Divide/1 -> lambda/1
  max calculation/1 -> max calculation1/1
  max calculation1/1 -> Divide/2
  Sum/1 -> Divide/1

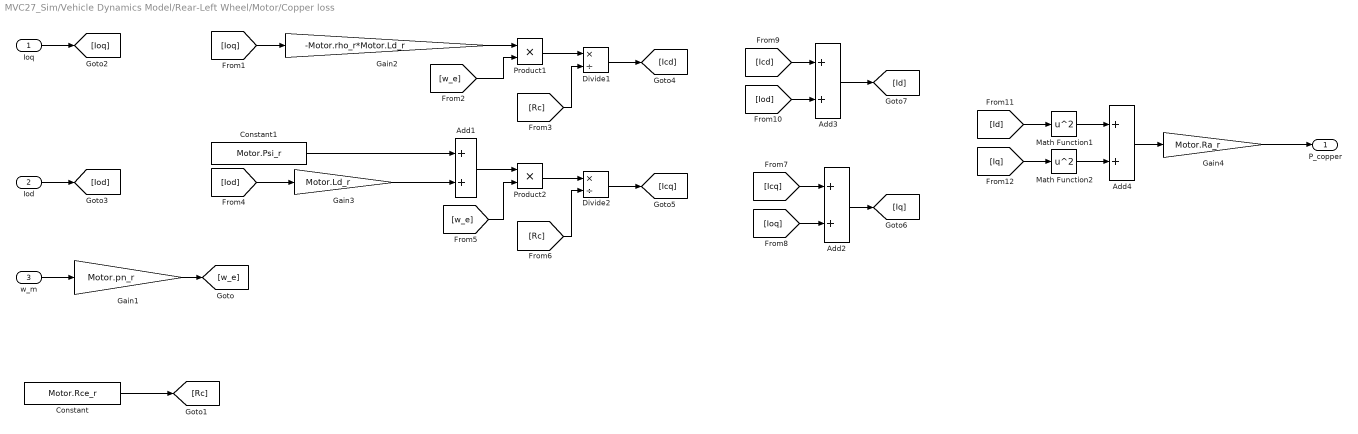
== system MVC27_Sim/Vehicle Dynamics Model/Rear-Left Wheel/Motor/Copper loss ==
  Ioq : Inport
  Iod : Inport  Port=2
  w_m : Inport  Port=3
  Add{1..4} (4 alike) : Sum
  Constant : Constant  Value=Motor.Rce_r
  Constant1 : Constant  Value=Motor.Psi_r
  Divide1 : Product  Inputs=*/
  Divide2 : Product  Inputs=*/
  Gain1 : Gain  Gain=Motor.pn_r
  Gain2 : Gain  Gain=-Motor.rho_r*Motor.Ld_r
  Gain3 : Gain  Gain=Motor.Ld_r
  Gain4 : Gain  Gain=Motor.Ra_r
  Math Function1 : Math  Operator=square  SignedPower=on
  Math Function2 : Math  Operator=square  SignedPower=on
  Product1 : Product
  Product2 : Product
  P_copper : Outport
  wires:
  w_m/1 -> Gain1/1
  Gain1/1 -> [w_e]
  Ioq/1 -> [Ioq]
  Iod/1 -> [Iod]
  [Ioq] -> Gain2/1
  Gain2/1 -> Product1/1
  [w_e] -> Product1/2
  Product1/1 -> Divide1/1
  [Rc] -> Divide1/2
  Divide1/1 -> [Icd]
  Constant1/1 -> Add1/1
  [Iod] -> Gain3/1
  Gain3/1 -> Add1/2
  Add1/1 -> Product2/1
  [w_e] -> Product2/2
  Product2/1 -> Divide2/1
  [Rc] -> Divide2/2
  Divide2/1 -> [Icq]
  [Icq] -> Add2/1
  [Ioq] -> Add2/2
  Add2/1 -> [Iq]
  [Icd] -> Add3/1
  Add3/1 -> [Id]
  [Iod] -> Add3/2
  [Id] -> Math Function1/1
  [Iq] -> Math Function2/1
  Math Function1/1 -> Add4/1
  Math Function2/1 -> Add4/2
  Add4/1 -> Gain4/1
  Gain4/1 -> P_copper/1
  Constant/1 -> [Rc]

== system MVC27_Sim/Vehicle Dynamics Model/Rear-Left Wheel/Motor/Iq_cal ==
  trq : Inport
  Psi_eq : Inport  Port=2
  Divide : Product  Inputs=*/
  Gain : Gain  Gain=Motor.pn_r
  Ioq : Outport
  wires:
  Psi_eq/1 -> Gain/1
  Divide/1 -> Ioq/1
  Gain/1 -> Divide/2
  trq/1 -> Divide/1

== system MVC27_Sim/Vehicle Dynamics Model/Rear-Left Wheel/Motor/Iron loss ==
  Ioq : Inport
  Iod : Inport  Port=2
  w_m : Inport  Port=3
  Add1 : Sum
  Add4 : Sum
  Constant : Constant  Value=Motor.Rce_r
  Constant1 : Constant  Value=Motor.Psi_r
  Divide1 : Product  Inputs=*/
  Divide2 : Product  Inputs=*/
  Gain1 : Gain  Gain=Motor.pn_r
  Gain2 : Gain  Gain=-Motor.rho_r*Motor.Ld_r
  Gain3 : Gain  Gain=Motor.Ld_r
  Math Function1 : Math  Operator=square  SignedPower=on
  Math Function2 : Math  Operator=square  SignedPower=on
  Product1 : Product
  Product2 : Product
  Product3 : Product
  P_iron : Outport
  wires:
  Gain1/1 -> [w_e]
  w_m/1 -> Gain1/1
  [Rc] -> Divide2/2
  Constant1/1 -> Add1/1
  Gain3/1 -> Add1/2
  Add1/1 -> Product2/1
  Divide1/1 -> [Icd]
  Product1/1 -> Divide1/1
  [Iod] -> Gain3/1
  Gain2/1 -> Product1/1
  Divide2/1 -> [Icq]
  [Rc] -> Divide1/2
  [Ioq] -> Gain2/1
  [w_e] -> Product2/2
  [w_e] -> Product1/2
  Product2/1 -> Divide2/1
  Ioq/1 -> [Ioq]
  Iod/1 -> [Iod]
  [Icd] -> Math Function1/1
  Math Function1/1 -> Add4/1
  [Icq] -> Math Function2/1
  Math Function2/1 -> Add4/2
  Add4/1 -> Product3/1
  [Rc] -> Product3/2
  Product3/1 -> P_iron/1
  Constant/1 -> [Rc]

== system MVC27_Sim/Vehicle Dynamics Model/Rear-Left Wheel/Motor/Output power ==
  trq : Inport
  w_m : Inport  Port=2
  Product : Product
  P_out : Outport
  wires:
  trq/1 -> Product/1
  w_m/1 -> Product/2
  Product/1 -> P_out/1

== system MVC27_Sim/Vehicle Dynamics Model/Rear-Left Wheel/Motor/Psi_eq ==
  Iod : Inport
  Add : Sum
  Constant : Constant  Value=Motor.Psi_r
  Gain4 : Gain  Gain=(1-Motor.rho_r)*Motor.Ld_r  SaturateOnIntegerOverflow=on  OutDataTypeStr=Inherit: Same as input  ParamDataTypeStr=Inherit: Same as input
  Psi_eq : Outport
  wires:
  Iod/1 -> Gain4/1
  Gain4/1 -> Add/2
  Constant/1 -> Add/1
  Add/1 -> Psi_eq/1

== system MVC27_Sim/Vehicle Dynamics Model/Rear-Left Wheel/Tire force model/Slip ratio calculation ==
  V : Inport
  Vw : Inport  Port=2
  Divide : Product  Inputs=*/
  Sum : Sum  Inputs=-+
  max calculation : MinMax  Function=max  Inputs=2
  max calculation1 : MinMax  Function=max  Inputs=2
  small number for anti division by zero : Constant  Value=eps
  lambda : Outport
  wires:
  small number for anti division by zero/1 -> max calculation1/2
  Vw/1 -> max calculation/2, Sum/2
  V/1 -> max calculation/1, Sum/1
  Divide/1 -> lambda/1
  max calculation/1 -> max calculation1/1
  max calculation1/1 -> Divide/2
  Sum/1 -> Divide/1

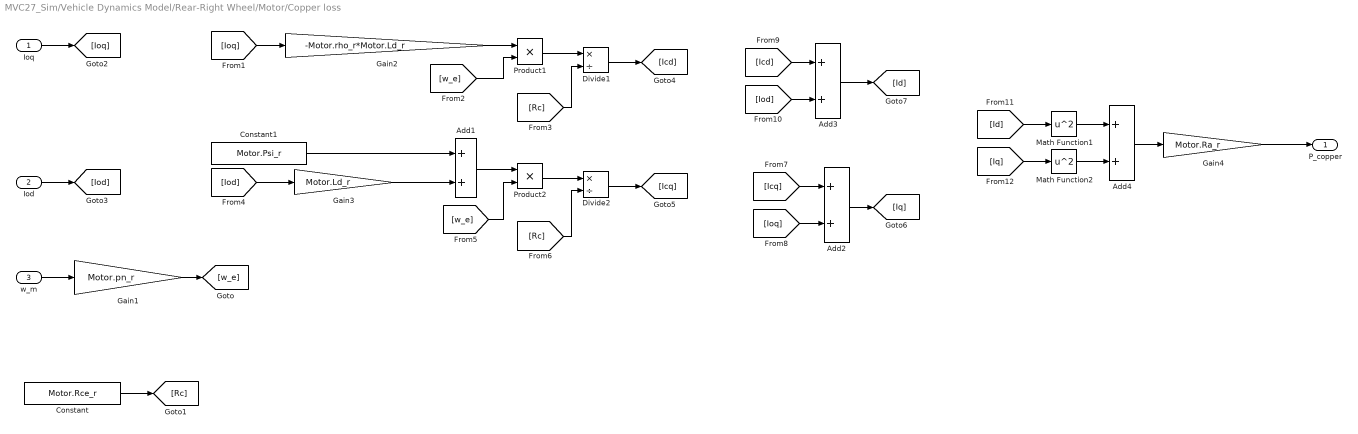
== system MVC27_Sim/Vehicle Dynamics Model/Rear-Right Wheel/Motor/Copper loss ==
  Ioq : Inport
  Iod : Inport  Port=2
  w_m : Inport  Port=3
  Add{1..4} (4 alike) : Sum
  Constant : Constant  Value=Motor.Rce_r
  Constant1 : Constant  Value=Motor.Psi_r
  Divide1 : Product  Inputs=*/
  Divide2 : Product  Inputs=*/
  Gain1 : Gain  Gain=Motor.pn_r
  Gain2 : Gain  Gain=-Motor.rho_r*Motor.Ld_r
  Gain3 : Gain  Gain=Motor.Ld_r
  Gain4 : Gain  Gain=Motor.Ra_r
  Math Function1 : Math  Operator=square  SignedPower=on
  Math Function2 : Math  Operator=square  SignedPower=on
  Product1 : Product
  Product2 : Product
  P_copper : Outport
  wires:
  w_m/1 -> Gain1/1
  Gain1/1 -> [w_e]
  Ioq/1 -> [Ioq]
  Iod/1 -> [Iod]
  [Ioq] -> Gain2/1
  Gain2/1 -> Product1/1
  [w_e] -> Product1/2
  Product1/1 -> Divide1/1
  [Rc] -> Divide1/2
  Divide1/1 -> [Icd]
  Constant1/1 -> Add1/1
  [Iod] -> Gain3/1
  Gain3/1 -> Add1/2
  Add1/1 -> Product2/1
  [w_e] -> Product2/2
  Product2/1 -> Divide2/1
  [Rc] -> Divide2/2
  Divide2/1 -> [Icq]
  [Icq] -> Add2/1
  [Ioq] -> Add2/2
  Add2/1 -> [Iq]
  [Icd] -> Add3/1
  Add3/1 -> [Id]
  [Iod] -> Add3/2
  [Id] -> Math Function1/1
  [Iq] -> Math Function2/1
  Math Function1/1 -> Add4/1
  Math Function2/1 -> Add4/2
  Add4/1 -> Gain4/1
  Gain4/1 -> P_copper/1
  Constant/1 -> [Rc]

== system MVC27_Sim/Vehicle Dynamics Model/Rear-Right Wheel/Motor/Iq_cal ==
  trq : Inport
  Psi_eq : Inport  Port=2
  Divide : Product  Inputs=*/
  Gain : Gain  Gain=Motor.pn_r
  Ioq : Outport
  wires:
  Gain/1 -> Divide/2
  Divide/1 -> Ioq/1
  Psi_eq/1 -> Gain/1
  trq/1 -> Divide/1

== system MVC27_Sim/Vehicle Dynamics Model/Rear-Right Wheel/Motor/Iron loss ==
  Ioq : Inport
  Iod : Inport  Port=2
  w_m : Inport  Port=3
  Add1 : Sum
  Add4 : Sum
  Constant : Constant  Value=Motor.Rce_r
  Constant1 : Constant  Value=Motor.Psi_r
  Divide1 : Product  Inputs=*/
  Divide2 : Product  Inputs=*/
  Gain1 : Gain  Gain=Motor.pn_r
  Gain2 : Gain  Gain=-Motor.rho_r*Motor.Ld_r
  Gain3 : Gain  Gain=Motor.Ld_r
  Math Function1 : Math  Operator=square  SignedPower=on
  Math Function2 : Math  Operator=square  SignedPower=on
  Product1 : Product
  Product2 : Product
  Product3 : Product
  P_iron : Outport
  wires:
  Gain1/1 -> [w_e]
  w_m/1 -> Gain1/1
  [Rc] -> Divide2/2
  Constant1/1 -> Add1/1
  Gain3/1 -> Add1/2
  Add1/1 -> Product2/1
  Divide1/1 -> [Icd]
  Product1/1 -> Divide1/1
  [Iod] -> Gain3/1
  Gain2/1 -> Product1/1
  Divide2/1 -> [Icq]
  [Rc] -> Divide1/2
  [Ioq] -> Gain2/1
  [w_e] -> Product2/2
  [w_e] -> Product1/2
  Product2/1 -> Divide2/1
  Ioq/1 -> [Ioq]
  Iod/1 -> [Iod]
  [Icd] -> Math Function1/1
  Math Function1/1 -> Add4/1
  [Icq] -> Math Function2/1
  Math Function2/1 -> Add4/2
  Add4/1 -> Product3/1
  [Rc] -> Product3/2
  Product3/1 -> P_iron/1
  Constant/1 -> [Rc]

== system MVC27_Sim/Vehicle Dynamics Model/Rear-Right Wheel/Motor/Output power ==
  trq : Inport
  w_m : Inport  Port=2
  Product : Product
  P_out : Outport
  wires:
  trq/1 -> Product/1
  w_m/1 -> Product/2
  Product/1 -> P_out/1

== system MVC27_Sim/Vehicle Dynamics Model/Rear-Right Wheel/Motor/Psi_eq ==
  Iod : Inport
  Add : Sum
  Constant : Constant  Value=Motor.Psi_r
  Gain4 : Gain  Gain=(1-Motor.rho_r)*Motor.Ld_r  SaturateOnIntegerOverflow=on  OutDataTypeStr=Inherit: Same as input  ParamDataTypeStr=Inherit: Same as input
  Psi_eq : Outport
  wires:
  Iod/1 -> Gain4/1
  Gain4/1 -> Add/2
  Constant/1 -> Add/1
  Add/1 -> Psi_eq/1

== system MVC27_Sim/Vehicle Dynamics Model/Rear-Right Wheel/Tire force model/Slip ratio calculation ==
  V : Inport
  Vw : Inport  Port=2
  Divide : Product  Inputs=*/
  Sum : Sum  Inputs=-+
  max calculation : MinMax  Function=max  Inputs=2
  max calculation1 : MinMax  Function=max  Inputs=2
  small number for anti division by zero : Constant  Value=eps
  lambda : Outport
  wires:
  small number for anti division by zero/1 -> max calculation1/2
  Vw/1 -> max calculation/2, Sum/2
  V/1 -> max calculation/1, Sum/1
  Divide/1 -> lambda/1
  max calculation/1 -> max calculation1/1
  max calculation1/1 -> Divide/2
  Sum/1 -> Divide/1

== matlab function MVC27_Sim/Scope/Energy calculation/Longitudinal misalignment ==
  data: u input; y output
function y = fcn(u)
N = 500;
delta = -0.4;
if (u <= 500.1)
    delta = -0.4;
end;
if (u >= 1498.9)
    delta = 0.4;
end;
if (u > 500.1) && (u < 1498.9)
    for i = 1:N
        Pos_coil = 500.5 + 2*(i-1);
        delta_x = u - Pos_coil;
        if (abs(delta_x) < 0.4)
            delta = delta_x;
        end;
    end;
end;
y = delta;

== matlab function MVC27_Sim/Vehicle Dynamics Model/Velocity and Slip Angle of Wheels ==
  data: V_fr output; V_fl output; V_rr output; V_rl output; alpha_fr output; delta_f input; alpha_fl output; alpha_rr output; beta input; V input; gamma input; delta_r input; df input; dr input; lf input; lr input; alpha_rl output
function [V_fr,V_fl,V_rr,V_rl,alpha_fr,alpha_fl,alpha_rr,alpha_rl] = fcn(delta_f,beta,V,gamma,delta_r,df,dr,lf,lr)
    V_fl = sqrt((V*sin(beta)+gamma*lf)^2+(V*cos(beta)-gamma*df/2)^2);
    V_fr = sqrt((V*sin(beta)+gamma*lf)^2+(V*cos(beta)+gamma*df/2)^2);
    V_rl = sqrt((V*sin(beta)-gamma*lr)^2+(V*cos(beta)-gamma*dr/2)^2);
    V_rr = sqrt((V*sin(beta)-gamma*lr)^2+(V*cos(beta)+gamma*dr/2)^2);
    
    alpha_fl = atan((V*sin(beta)+gamma*lf)/(V*cos(beta)-gamma*df/2))-delta_f;
    alpha_fr = atan((V*sin(beta)+gamma*lf)/(V*cos(beta)+gamma*df/2))-delta_f;
    alpha_rl = atan((V*sin(beta)-gamma*lr)/(V*cos(beta)-gamma*dr/2))-delta_r;
    alpha_rr = atan((V*sin(beta)-gamma*lr)/(V*cos(beta)+gamma*dr/2))-delta_r;

== matlab function MVC27_Sim/Scope/Energy calculation/DWPT efficiency map ==
  data: u1 input; y output; u2 input
function y = fcn(u1,u2)
%
% u1: longitudinal misalignment, u2: lateral misalignment

% DWPT circuit
WPT.freq = 85000;          % Frequency of the inverter [Hz]
WPT.L1 = 142.326e-6;       % GA coil inductance [H]
WPT.L2 = 54.2047e-6;       % VA coil inductance [H]
WPT.R1 = 85.02/1000;       % GA coil resistance [Ohm]
WPT.R2 = 39.88/1000;       % VA coil resistance [Ohm]
% Mutual inductance map
xx = [-400 -350 -300 -250 -200 -150 -100 -50 0 50 100 150 200 250 300 350 400]; % longitudinal misalignment [mm]
yy = [-150 -100 -50 0 50 100 150]; % lateral misalignment [mm]
z000 = [18.366 18.12075 18.2285 18.62175 19.4505 22.78625 21.99725 18.1625 12.584]; 
z050 = [16.16075 15.495 15.44675 15.71575 18.70275 19.3575 18.8615 15.5565 10.6605];
z100 = [9.85675 9.60925 10.05325 10.28375 11.30575 13.352 13.16575 10.59525 6.935];
z150 = [4.81875 4.1325 4.1535 5.24425 6.22225 7.28925 6.64025 5.4515 3.44175];
%
z000f = flip(z000); z050f = flip(z050); z100f = flip(z100); z150f = flip(z150); 
z000f(9) = []; z050f(9) = []; z100f(9) = []; z150f(9) = [];
%
zz = [z150f z150;          % Mutual inductance [uH]
     z100f z100;
     z050f z050;
     z000f z000;
     z050f z050;
     z100f z100;
     z150f z150];
%
eta_wpt = 0;              % effciency
w = 2*pi*WPT.freq;        % inverter frequency
Q1 = w*WPT.L1/WPT.R1;     % Q factor of GA coil
Q2 = w*WPT.L2/WPT.R2;     % Q factor of VA coil
Lm = 0;                   % mutual inductance
k = 0;                    % coupling coefficient
%
% If the misalignment is too big, 
% the DWPT system neglects to transfer energy
if (abs(u1) > 380) || (abs(u2) > 70) 
    eta_wpt = 0;
end;
% DWPT system operates if 
% the misalignments are less than certain thresholds
if (abs(u1) <= 380) && (abs(u2) <= 70) 
    Lm = (1e-6)*interp2(xx, yy, zz, u1, u2);
    k = Lm/sqrt(WPT.L1*WPT.L2);
    eta_wpt = k*k*Q1*Q2/((1+sqrt(1+Q1*Q2*k*k))^2);
end;
%
y = eta_wpt;  % efficiency
